simulink model "modelo_1_linear"  (R2026a)
settings: Solver=ode45  StopTime=8
libraries: cstblocks_lti x1

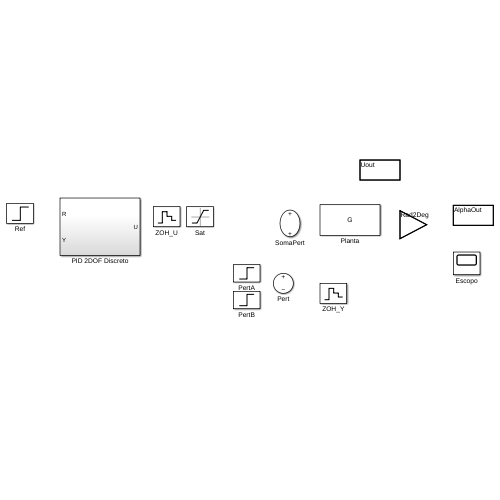
[thumbnail: Simulink's stored preview of the top-level diagram]
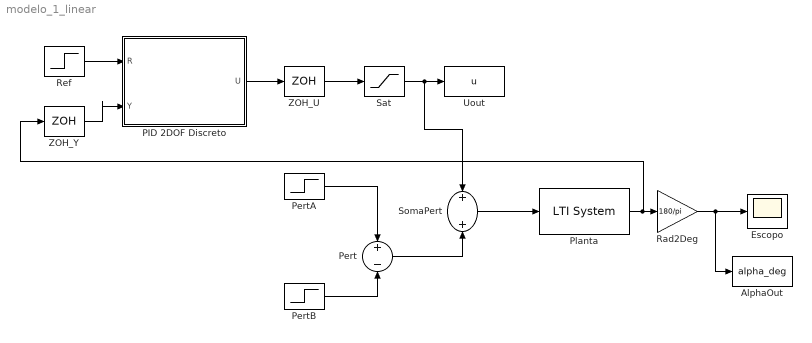
== system modelo_1_linear ==
  AlphaOut : ToWorkspace  VariableName=alpha_deg  SaveFormat=Timeseries  SampleTime=-1
  Escopo : Scope
  PID 2DOF Discreto : Subsystem
  Pert : Sum  Inputs=+-
  PertA : Step  Time=2  FinalValue=60  SampleTime=0
  PertB : Step  Time=2.3  FinalValue=60  SampleTime=0
  Planta : cstblocks_lti/LTI System  sys=G  IC=[]  PadeOrder=0
      settings: LibrarySourceBlock=cstblocks/LTI System
  Rad2Deg : Gain  Gain=180/pi
  Ref : Step  Time=0  FinalValue=0  SampleTime=0
  Sat : Saturate  UpperLimit=255  LowerLimit=-255
  SomaPert : Sum
  Uout : ToWorkspace  VariableName=u  SaveFormat=Timeseries  SampleTime=-1
  ZOH_U : ZeroOrderHold  SampleTime=0.02
  ZOH_Y : ZeroOrderHold  SampleTime=0.02
  wires:
  Planta/1 -> Rad2Deg/1, ZOH_Y/1
  SomaPert/1 -> Planta/1
  Pert/1 -> SomaPert/2
  Sat/1 -> Uout/1, SomaPert/1
  PertB/1 -> Pert/2
  PertA/1 -> Pert/1
  ZOH_U/1 -> Sat/1
  PID 2DOF Discreto/1(U) -> ZOH_U/1
  Rad2Deg/1 -> Escopo/1, AlphaOut/1
  ZOH_Y/1 -> PID 2DOF Discreto/2(Y)
  Ref/1 -> PID 2DOF Discreto/1(R)

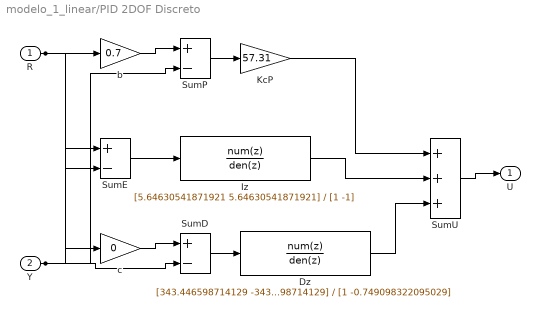
== system modelo_1_linear/PID 2DOF Discreto ==
  R : Inport
  Y : Inport  Port=2
  Dz : DiscreteTransferFcn  Numerator=[343.446598714129 -343.446598714129]  Denominator=[1 -0.749098322095029]  SampleTime=0.02
  Iz : DiscreteTransferFcn  Numerator=[5.64630541871921 5.64630541871921]  Denominator=[1 -1]  SampleTime=0.02
  KcP : Gain  Gain=57.31
  SumD : Sum  Inputs=+-
  SumE : Sum  Inputs=+-
  SumP : Sum  Inputs=+-
  SumU : Sum  Inputs=+++
  b : Gain  Gain=0.7
  c : Gain  Gain=0
  U : Outport
  wires:
  R/1 -> b/1, SumE/1, c/1
  b/1 -> SumP/1
  Y/1 -> SumP/2, SumE/2, SumD/2
  SumP/1 -> KcP/1
  SumE/1 -> Iz/1
  c/1 -> SumD/1
  SumD/1 -> Dz/1
  KcP/1 -> SumU/1
  Iz/1 -> SumU/2
  Dz/1 -> SumU/3
  SumU/1 -> U/1
